simulink model "gncc_uav_toolbox"  (R2025b)
settings: Solver=ode45  StartTime=0  StopTime=cfg.stopTime  MaxStep=0.01  RelTol=1e-5
undefined symbols (not defined in the file or in its folder): C, cfg, entryPoint, homeAir, lastPoint, searchW
libraries: uavalgslib x2, uavutilslib x1
settings Model: Creator=andrei  LastModifiedBy=andrei

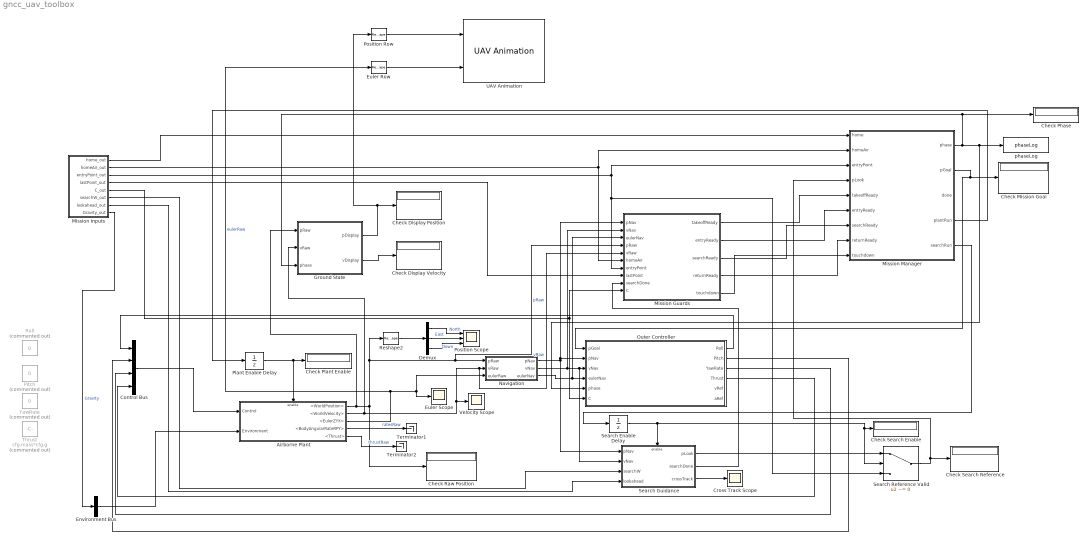
== system gncc_uav_toolbox ==
  Airborne Plant : Subsystem
      settings: MinAlgLoopOccurrences=on
  Check Display Position : Display
  Check Display Velocity : Display
  Check Mission Goal : Display
  Check Phase : Display
  Check Plant Enable : Display
  Check Raw Position : Display
  Check Search Enable : Display
  Check Search Reference : Display
  Control Bus : BusCreator  Inputs=4  OutDataTypeStr=Bus: GNControlBus  NonVirtualBus=on
  Cross Track Scope : Scope
      settings: DataLoggingVariableName=ScopeData3
  Demux : Demux  Outputs=3
  Environment Bus : BusCreator  Inputs=1  OutDataTypeStr=Bus: GNEnvironmentBus  NonVirtualBus=on
  Euler Row : Reshape  OutputDimensionality=Customize  OutputDimensions=[1 3]
  Euler Scope : Scope
      settings: DataLoggingVariableName=ScopeData2
  Ground State : MATLAB Function  TreatAsAtomicUnit=on
  Mission Guards : MATLAB Function  TreatAsAtomicUnit=on
  Mission Inputs : Subsystem
  Mission Manager : Stateflow chart  TreatAsAtomicUnit=on
  Navigation : Subsystem
  Outer Controller : Subsystem
  Pitch : Constant  Commented=on  Value=0  VectorParams1D=off
  Plant Enable Delay : UnitDelay  InitialCondition=false  SampleTime=cfg.ctrlTs  HasFrameUpgradeWarning=on
  Position Row : Reshape  OutputDimensionality=Customize  OutputDimensions=[1 3]
  Position Scope : Scope  NumInputPorts=3
      settings: ActiveDisplayYMinimum=-36.831864712326947  ActiveDisplayYMaximum=14.10248446170346
  Reshape2 : Reshape
  Roll : Constant  Commented=on  Value=0  VectorParams1D=off
  Search Guidance : Subsystem  TreatAsAtomicUnit=on
  Search Enable Delay : UnitDelay  InitialCondition=false  SampleTime=cfg.ctrlTs  HasFrameUpgradeWarning=on
  Search Reference Valid : Switch  Criteria=u2 ~= 0  SaturateOnIntegerOverflow=off  InputSameDT=off
  Terminator1 : Terminator
  Terminator2 : Terminator
  Thrust : Constant  Commented=on  Value=cfg.mass*cfg.g  VectorParams1D=off
  UAV Animation : uavutilslib/UAV Animation  NumUAV=1  DynamicUAVConfig=off  UAVType=Multirotor  UAVSize=0.3  UAVColor=[0 0.45 0.74]  UAVTrajectoryAlpha=1  InertialZDirection=Down  RotationFormat=Euler ZYX  DrawMarkers=off  SampleTime=cfg.animTs
  Velocity Scope : Scope
      settings: ActiveDisplayYMinimum=-2.4801881496796212  ActiveDisplayYMaximum=2.1396138851515727
  YawRate : Constant  Commented=on  Value=0  VectorParams1D=off
  phaseLog : ToWorkspace  VariableName=phaseLog  SaveFormat=Timeseries  SampleTime=cfg.ctrlTs
  wires:
  Navigation/1(pNav) -> Search Guidance/1(pNav), Mission Guards/1(pNav), Outer Controller/2(pNav)
  Navigation/2(vNav) -> Mission Guards/2(vNav), Search Guidance/2(vNav), Outer Controller/3(vNav)
  Navigation/3(eulerNav) -> Mission Guards/3(eulerNav), Outer Controller/4(eulerNav)
  Outer Controller/1(Roll) -> Control Bus/1
  Outer Controller/2(Pitch) -> Control Bus/2
  Outer Controller/3(YawRate) -> Control Bus/3
  Outer Controller/4(Thrust) -> Control Bus/4
  Reshape2/1 -> Demux/1
  Demux/1 -> Position Scope/1  "North"
  Demux/2 -> Position Scope/2  "East"
  Demux/3 -> Position Scope/3  "Down"
  Search Enable Delay/1 -> Search Reference Valid/2, Check Search Enable/1, Search Guidance/Enable
  Search Guidance/1(pLook) -> Search Reference Valid/1
  Search Guidance/2(searchDone) -> Mission Guards/9(searchDone)
  Mission Guards/1(takeoffReady) -> Mission Manager/5(takeoffReady)
  Mission Guards/2(entryReady) -> Mission Manager/6(entryReady)
  Mission Guards/3(searchReady) -> Mission Manager/7(searchReady)
  Mission Guards/4(returnReady) -> Mission Manager/8(returnReady)
  Mission Guards/5(touchdown) -> Mission Manager/9(touchdown)
  Airborne Plant/2(<WorldVelocity>) -> Ground State/2(vRaw), Mission Guards/5(vRaw), Navigation/2(vRaw), Velocity Scope/1  "vRaw"
  Airborne Plant/3(<EulerZYX>) -> Euler Row/1, Euler Scope/1, Navigation/3(eulerRaw)  "eulerRaw"
  Airborne Plant/1(<WorldPosition>) -> Ground State/1(pRaw), Check Raw Position/1, Mission Guards/4(pRaw), Navigation/1(pRaw), Reshape2/1  "pRaw"
  Control Bus/1 -> Airborne Plant/1(Control)
  Environment Bus/1 -> Airborne Plant/2(Environment)
  Airborne Plant/4(<BodyAngularRateRPY>) -> Terminator1/1  "ratesRaw"
  Airborne Plant/5(<Thrust>) -> Terminator2/1  "thrustRaw"
  Plant Enable Delay/1 -> Check Plant Enable/1, Airborne Plant/Enable
  Mission Manager/4(plantRun) -> Plant Enable Delay/1
  Mission Manager/5(searchRun) -> Search Enable Delay/1
  Search Reference Valid/1 -> Check Search Reference/1, Mission Manager/4(pLook)
  Mission Manager/1(phase) -> phaseLog/1, Outer Controller/5(phase), Check Phase/1, Ground State/3(phase)
  Ground State/2(vDisplay) -> Check Display Velocity/1
  Ground State/1(pDisplay) -> Position Row/1, Check Display Position/1
  Mission Manager/2(pGoal) -> Check Mission Goal/1, Outer Controller/1(pGoal)
  Mission Inputs/2(homeAir_out) -> Mission Guards/6(homeAir), Mission Manager/2(homeAir)
  Mission Inputs/3(entryPoint_out) -> Mission Guards/7(entryPoint), Search Reference Valid/3, Mission Manager/3(entryPoint)
  Mission Inputs/5(C_out) -> Outer Controller/6(C), Mission Guards/10(C)
  Mission Inputs/1(home_out) -> Mission Manager/1(home)
  Mission Inputs/4(lastPoint_out) -> Mission Guards/8(lastPoint)
  Mission Inputs/6(searchW_out) -> Search Guidance/3(searchW)
  Mission Inputs/7(lookahead_out) -> Search Guidance/4(lookahead)
  Mission Inputs/8(Gravity_out) -> Environment Bus/1  "Gravity"
  Search Guidance/3(crossTrack) -> Cross Track Scope/1
  Position Row/1 -> UAV Animation/1
  Euler Row/1 -> UAV Animation/2

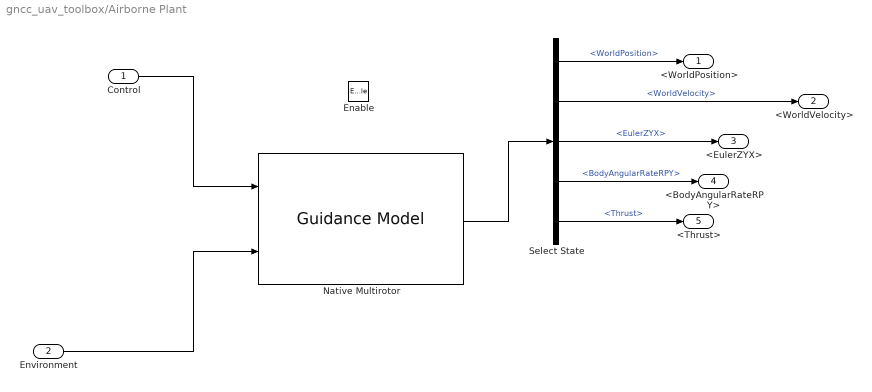
== system gncc_uav_toolbox/Airborne Plant ==
  Control : Inport
  Environment : Inport  Port=2
  Enable : EnablePort
  Native Multirotor : uavalgslib/Guidance Model  ModelType=MultirotorGuidance  NumInstances=1  SpecifiedDataType=double  SimulateUsing=Interpreted execution  InitialWorldPositionMultirotor=home  InitialWorldVelocityMultirotor=[0; 0; 0]  InitialEulerZYXMultirotor=[0; 0; 0]  InitialBodyAngularRateRPYMultirotor=[0; 0; 0]  InitialThrustMultirotor=cfg.mass*cfg.g  InitialNorthFixedWing=0  InitialEastFixedWing=0  InitialHeightFixedWing=0  InitialAirSpeedFixedWing=0  InitialHeadingAngleFixedWing=0  InitialFlightPathAngleFixedWing=0  InitialRollAngleFixedWing=0  InitialRollAngleRateFixedWing=0  PDRollMultirotor=[3402.97,116.67]  PDPitchMultirotor=[3402.97, 116.67]  PYawRateMultirotor=1950  PThrustMultirotor=3900  MassMultirotor=cfg.mass  PHeightFixedWing=3.9  PHeadingAngleFixedWing=3.9  PFlightPathAngleFixedWing=39  PDRollFixedWing=[3402.97, 116.67]  PAirSpeedFixedWing=1  FlightPathAngleLimitsFixedWing=[-pi/2, pi/2]  StateBusName='GNStateBus'  ControlBusName='GNControlBus'  EnvironmentBusName='GNEnvironmentBus'  DataType=double
  Select State : BusSelector  OutputSignals=WorldPosition,WorldVelocity,EulerZYX,BodyAngularRateRPY,Thrust
  <WorldPosition> : Outport
  <WorldVelocity> : Outport  Port=2
  <EulerZYX> : Outport  Port=3
  <BodyAngularRateRPY> : Outport  Port=4
  <Thrust> : Outport  Port=5
  wires:
  Select State/4 -> <BodyAngularRateRPY>/1  "<BodyAngularRateRPY>"
  Environment/1 -> Native Multirotor/2
  Select State/5 -> <Thrust>/1  "<Thrust>"
  Select State/1 -> <WorldPosition>/1  "<WorldPosition>"
  Native Multirotor/1 -> Select State/1
  Control/1 -> Native Multirotor/1
  Select State/3 -> <EulerZYX>/1  "<EulerZYX>"
  Select State/2 -> <WorldVelocity>/1  "<WorldVelocity>"

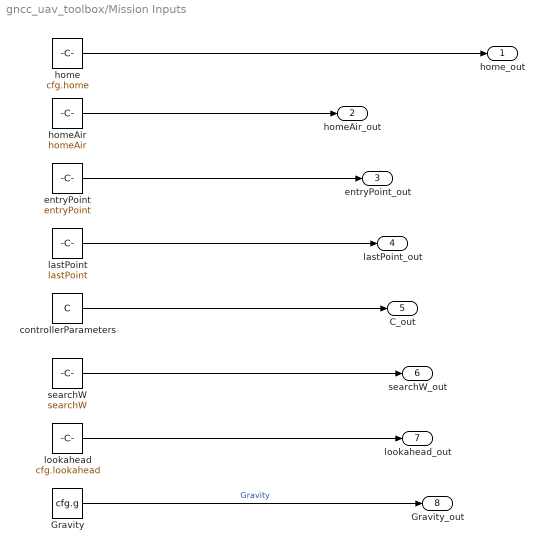
== system gncc_uav_toolbox/Mission Inputs ==
  Gravity : Constant  Value=cfg.g  VectorParams1D=off
  controllerParameters : Constant  Value=C
  entryPoint : Constant  Value=entryPoint  VectorParams1D=off
  home : Constant  Value=cfg.home  VectorParams1D=off
  homeAir : Constant  Value=homeAir  VectorParams1D=off
  lastPoint : Constant  Value=lastPoint  VectorParams1D=off
  lookahead : Constant  Value=cfg.lookahead
  searchW : Constant  Value=searchW
  home_out : Outport
  homeAir_out : Outport  Port=2
  entryPoint_out : Outport  Port=3
  lastPoint_out : Outport  Port=4
  C_out : Outport  Port=5
  searchW_out : Outport  Port=6
  lookahead_out : Outport  Port=7
  Gravity_out : Outport  Port=8
  wires:
  searchW/1 -> searchW_out/1
  lastPoint/1 -> lastPoint_out/1
  entryPoint/1 -> entryPoint_out/1
  lookahead/1 -> lookahead_out/1
  controllerParameters/1 -> C_out/1
  homeAir/1 -> homeAir_out/1
  Gravity/1 -> Gravity_out/1  "Gravity"
  home/1 -> home_out/1

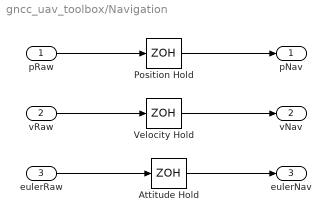
== system gncc_uav_toolbox/Navigation ==
  pRaw : Inport
  vRaw : Inport  Port=2
  eulerRaw : Inport  Port=3
  Attitude Hold : ZeroOrderHold  SampleTime=cfg.ctrlTs
  Position Hold : ZeroOrderHold  SampleTime=cfg.navTs
  Velocity Hold : ZeroOrderHold  SampleTime=cfg.navTs
  pNav : Outport
  vNav : Outport  Port=2
  eulerNav : Outport  Port=3
  wires:
  pRaw/1 -> Position Hold/1
  vRaw/1 -> Velocity Hold/1
  eulerRaw/1 -> Attitude Hold/1
  Position Hold/1 -> pNav/1
  Velocity Hold/1 -> vNav/1
  Attitude Hold/1 -> eulerNav/1

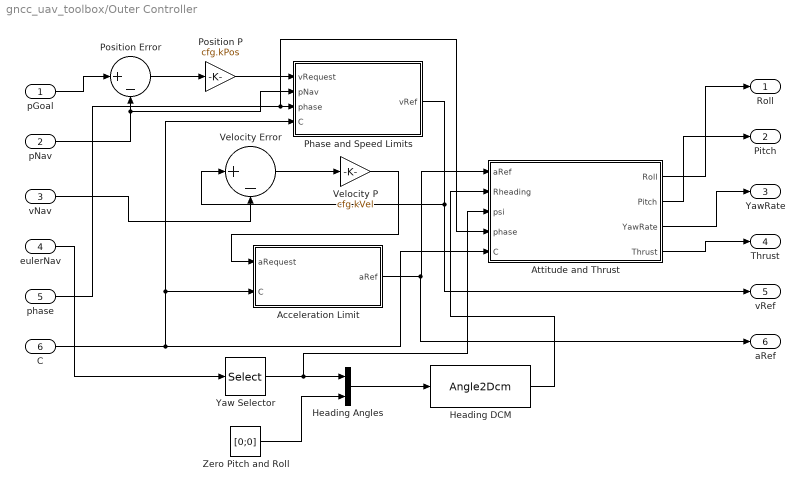
== system gncc_uav_toolbox/Outer Controller ==
  pGoal : Inport
  pNav : Inport  Port=2
  vNav : Inport  Port=3
  eulerNav : Inport  Port=4
  phase : Inport  Port=5
  C : Inport  Port=6
  Acceleration Limit : MATLAB Function  TreatAsAtomicUnit=on
  Attitude and Thrust : MATLAB Function  TreatAsAtomicUnit=on
  Heading Angles : Concatenate  Mode=Multidimensional array
  Heading DCM : Angle2Dcm
      settings: AttributesFormatString=Rotation Order: %<rotationOrder>
  Phase and Speed Limits : MATLAB Function  TreatAsAtomicUnit=on
  Position Error : Sum  Inputs=|+-
  Position P : Gain  Gain=cfg.kPos
  Velocity Error : Sum  Inputs=|+-
  Velocity P : Gain  Gain=cfg.kVel
  Yaw Selector : Selector  InputPortWidth=3  IndexOptions=Index vector (dialog)  Indices=[1]  OutputSizes=1
  Zero Pitch and Roll : Constant  Value=[0;0]  VectorParams1D=off
  Roll : Outport
  Pitch : Outport  Port=2
  YawRate : Outport  Port=3
  Thrust : Outport  Port=4
  vRef : Outport  Port=5
  aRef : Outport  Port=6
  wires:
  pGoal/1 -> Position Error/1
  pNav/1 -> Phase and Speed Limits/2(pNav), Position Error/2
  Phase and Speed Limits/1(vRef) -> vRef/1, Velocity Error/1
  vNav/1 -> Velocity Error/2
  Position Error/1 -> Position P/1
  Position P/1 -> Phase and Speed Limits/1(vRequest)
  phase/1 -> Attitude and Thrust/4(phase), Phase and Speed Limits/3(phase)
  C/1 -> Attitude and Thrust/5(C), Acceleration Limit/2(C), Phase and Speed Limits/4(C)
  Velocity Error/1 -> Velocity P/1
  Velocity P/1 -> Acceleration Limit/1(aRequest)
  Acceleration Limit/1(aRef) -> Attitude and Thrust/1(aRef), aRef/1
  eulerNav/1 -> Yaw Selector/1
  Yaw Selector/1 -> Attitude and Thrust/3(psi), Heading Angles/1
  Zero Pitch and Roll/1 -> Heading Angles/2
  Heading Angles/1 -> Heading DCM/1
  Heading DCM/1 -> Attitude and Thrust/2(Rheading)
  Attitude and Thrust/1(Roll) -> Roll/1
  Attitude and Thrust/2(Pitch) -> Pitch/1
  Attitude and Thrust/3(YawRate) -> YawRate/1
  Attitude and Thrust/4(Thrust) -> Thrust/1

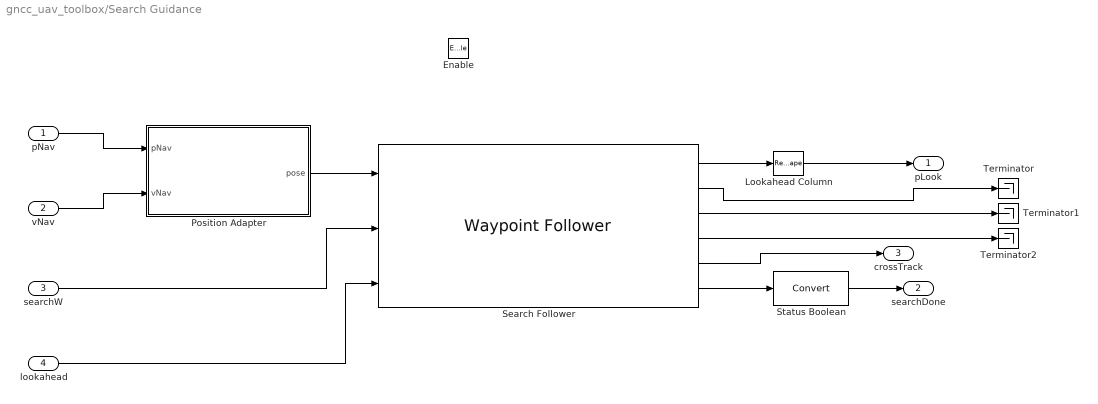
== system gncc_uav_toolbox/Search Guidance ==
  pNav : Inport
  vNav : Inport  Port=2
  searchW : Inport  Port=3
  lookahead : Inport  Port=4
  Enable : EnablePort
  Lookahead Column : Reshape  OutputDimensionality=Column vector (2-D)
  Position Adapter : MATLAB Function  TreatAsAtomicUnit=on
  Search Follower : uavalgslib/Waypoint Follower  UAVType=multirotor  StartFrom=first  TransitionRadiusSource=internal  TransitionRadius=cfg.transitionRadius  MinLookaheadDistance=0.1  HoverAtLastWaypoint=on  YawInput=off  ShowCrossTrackErrorOutput=on  ShowStatusOutput=on  SimulateUsing=Interpreted execution
  Status Boolean : DataTypeConversion  SaturateOnIntegerOverflow=off  RndMeth=Floor
  Terminator : Terminator
  Terminator1 : Terminator
  Terminator2 : Terminator
  pLook : Outport  OutputWhenDisabled=reset  InitialOutput=[0;0;0]
  searchDone : Outport  Port=2  OutputWhenDisabled=reset  InitialOutput=[false]
  crossTrack : Outport  Port=3  OutputWhenDisabled=reset  InitialOutput=[0]
  wires:
  pNav/1 -> Position Adapter/1(pNav)
  vNav/1 -> Position Adapter/2(vNav)
  Position Adapter/1(pose) -> Search Follower/1
  searchW/1 -> Search Follower/2
  lookahead/1 -> Search Follower/3
  Search Follower/1 -> Lookahead Column/1
  Lookahead Column/1 -> pLook/1
  Search Follower/6 -> Status Boolean/1
  Status Boolean/1 -> searchDone/1
  Search Follower/5 -> crossTrack/1
  Search Follower/4 -> Terminator2/1
  Search Follower/3 -> Terminator1/1
  Search Follower/2 -> Terminator/1

== matlab function gncc_uav_toolbox/Ground State ==
  settings: updateMethod=DISCRETE  sampleTime=cfg.ctrlTs
  data: pRaw input; pDisplay output; vRaw input; phase input; vDisplay output
function [pDisplay,vDisplay] = groundState(pRaw,vRaw,phase)
% Position and velocity for display and landed reporting.

% Normally report the unmodified plant state.
pDisplay = pRaw;
vDisplay = vRaw;

% During PRECHECK or COMPLETE, report the vehicle on the ground.
if phase == 0 || phase == 6
    pDisplay(3) = 0;
    vDisplay = zeros(3,1);
end
end

== matlab function gncc_uav_toolbox/Outer Controller/Acceleration Limit ==
  data: aRequest input; aRef output; C input
function aRef = limitAcceleration(aRequest,C)

aRef=aRequest; s=norm(aRef);

if s>C(5)

    aRef=aRef*(C(5)/s);

end

end

== matlab function gncc_uav_toolbox/Outer Controller/Phase and Speed Limits ==
  settings: updateMethod=DISCRETE  sampleTime=cfg.ctrlTs
  data: vRequest input; vRef output; pNav input; phase input; C input
function vRef = limitVelocity(vRequest,pNav,phase,C)

vRef=vRequest;

if phase==0 || phase==6

    vRef=zeros(3,1);

elseif phase==1

    vRef(1:2)=0;

elseif phase==5

    vRef=zeros(3,1);

    vRef(3)=min(C(4),max(0.03,C(1)*max(0,-pNav(3))));

end

s=norm(vRef); limit=min(C(2),C(3));

if s>limit

    vRef=vRef*(limit/s);

end

end

== matlab function gncc_uav_toolbox/Outer Controller/Attitude and Thrust ==
  settings: updateMethod=DISCRETE  sampleTime=cfg.ctrlTs
  data: Roll output; Pitch output; YawRate output; Thrust output; aRef input; Rheading input; psi input; phase input; C input
function [Roll,Pitch,YawRate,Thrust] = accelToCommands(aRef,Rheading,psi,phase,C)

m=C(6); g=C(7); tiltMax=C(8);

aHeading=Rheading*aRef;

verticalSupport=max(0.5*g,g-aHeading(3));

supportNorm=sqrt(aHeading(1)^2+aHeading(2)^2+verticalSupport^2);

Roll=asin(max(-1,min(1,aHeading(2)/supportNorm)));

Pitch=atan2(-aHeading(1),verticalSupport);

Roll=max(-tiltMax,min(tiltMax,Roll));

Pitch=max(-tiltMax,min(tiltMax,Pitch));

Thrust=m*verticalSupport/max(0.2,cos(Roll)*cos(Pitch));

Thrust=max(0,min(2*m*g,Thrust));

YawRate=max(-0.3,min(0.3,-psi));

if phase==0 || phase==6

    Roll=0; Pitch=0; YawRate=0; Thrust=0;

end

end

== matlab function gncc_uav_toolbox/Search Guidance/Position Adapter ==
  data: pNav input; pose output; vNav input
function pose = makeFollowerPose(pNav,vNav)

if hypot(vNav(1),vNav(2))>1e-4

    chi=atan2(vNav(2),vNav(1));

else

    chi=0;

end

pose=[pNav;chi];

end

== matlab function gncc_uav_toolbox/Mission Guards ==
  settings: updateMethod=DISCRETE  sampleTime=cfg.ctrlTs
  data: pNav input; takeoffReady output; vNav input; eulerNav input; pRaw input; vRaw input; homeAir input; entryPoint input; lastPoint input; searchDone input; C input; entryReady output; searchReady output; returnReady output; touchdown output
function [takeoffReady,entryReady,searchReady,returnReady, touchdown] = missionGuards(pNav,vNav,eulerNav,pRaw,vRaw,homeAir, entryPoint,lastPoint,searchDone,C)
slow=norm(vNav)<=C(11);
takeoffReady=norm(pNav-homeAir)<=C(9) && slow;
entryReady=norm(pNav-entryPoint)<=C(9) && slow;
searchReady=searchDone && norm(pNav-lastPoint)<=C(9) && slow;
level=abs(eulerNav(2))<=deg2rad(1) && abs(eulerNav(3))<=deg2rad(1);
returnReady=norm(pNav-homeAir)<=C(10) && slow && level;
touchdown=pRaw(3)>=0 && vRaw(3)>=-0.02;
end

== stateflow chart gncc_uav_toolbox/Mission Manager ==
  settings: updateMethod=DISCRETE  sampleTime=cfg.ctrlTs
  state PRECHECK
    entry, during:
    phase=0;
    pGoal=home;
    done=false;
    plantRun=false;
    searchRun=false;
  state TRANSIT
    entry, during:
    phase=2;
    pGoal=entryPoint;
    done=false;
    plantRun=true;
    searchRun=false;
  state SEARCH
    entry, during:
    phase=3;
    pGoal=pLook;
    done=false;
    plantRun=true;
    searchRun=true;
  state TAKEOFF
    entry, during:
    phase=1;
    pGoal=homeAir;
    done=false;
    plantRun=true;
    searchRun=false;
  state RETURN
    entry, during:
    phase=4;
    pGoal=homeAir;
    done=false;
    plantRun=true;
    searchRun=false;
  state COMPLETE
    entry, during:
    phase=6;
    pGoal=home;
    done=true;
    plantRun=false;
    searchRun=false;
  state LAND
    entry, during:
    phase=5;
    pGoal=home;
    done=false;
    plantRun=true;
    searchRun=false;
  (default) -> PRECHECK
  PRECHECK -> TAKEOFF : after(1,sec)
  TAKEOFF -> TRANSIT : [takeoffReady]
  TRANSIT -> SEARCH : [entryReady]
  SEARCH -> RETURN : [searchReady]
  RETURN -> LAND : [returnReady]
  LAND -> COMPLETE : [touchdown]
  data: home input double size=[3, 1]; homeAir input double size=[3, 1]; entryPoint input double size=[3, 1]; pLook input double size=[3, 1]; takeoffReady input boolean size=1; entryReady input boolean size=1; searchReady input boolean size=1; returnReady input boolean size=1; touchdown input boolean size=1; phase output double size=1; pGoal output double size=[3, 1]; done output boolean size=1; plantRun output boolean size=1; searchRun output boolean size=1
